simulink model "test"  (R2024b)
settings: Solver=VariableStepAuto  StartTime=0.0  StopTime=0.2  FixedStep=1e-6  RelTol=1e-3
libraries: spsMosfetLib x12, spsDiodeLib x6, spsSeriesRLCBranchLib x6, spsCurrentMeasurementLib x3, spsDCVoltageSourceLib x3, spsVoltageMeasurementLib x3, spsSeriesRLCLoadLib x1, spspowerguiLib x1
settings Model: Creator=medos  LastModifiedBy=medos
settings DataIOCC: InspectSignalLogs=on  ReturnWorkspaceOutputs=off

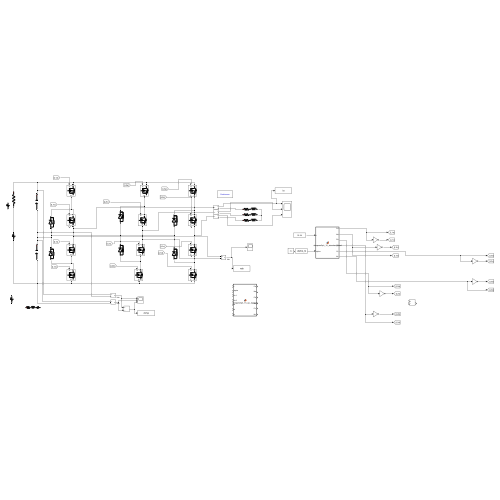
[thumbnail: Simulink's stored preview of the top-level diagram]
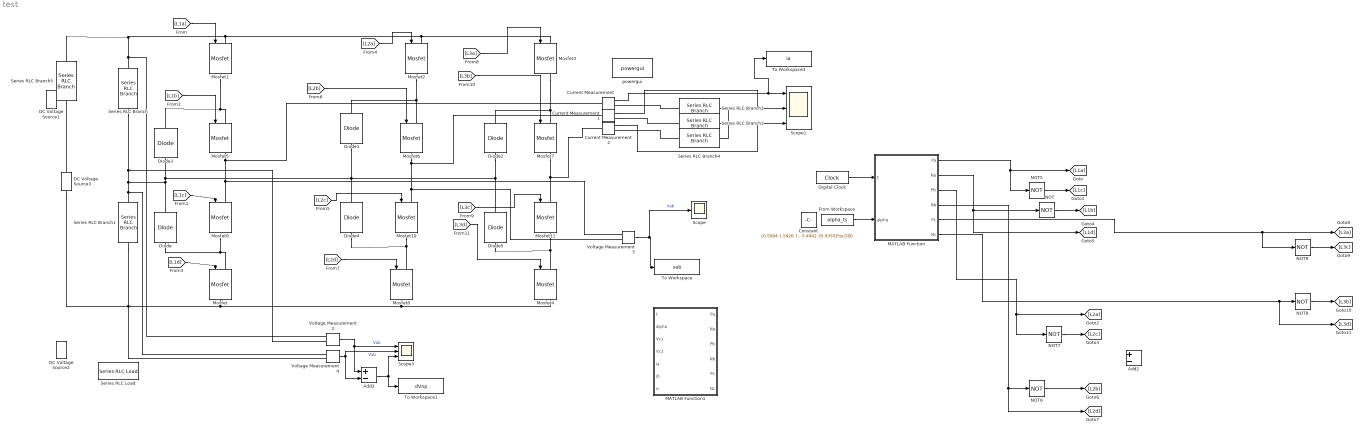
== system test ==
  Add2 : Sum  Inputs=+-
  Add3 : Sum  Inputs=+-
  Constant : Constant  Value="[0.5094\t1.5926\t7.8326\t9.5495\t13.4005\t15.2995\t15.5495\t16.5629\t19.0904\t22.9505\t24.7507\t29.3515\t30.4092\t35.4942\t35.9355]*pi/180"  SampleTime=-1
  Current Measurement : spsCurrentMeasurementLib/Current Measurement  PhasorSimulation=off  OutputType=Complex  PSBequivalent=0
  Current Measurement1 : spsCurrentMeasurementLib/Current Measurement  PhasorSimulation=off  OutputType=Complex  PSBequivalent=0
  Current Measurement2 : spsCurrentMeasurementLib/Current Measurement  PhasorSimulation=off  OutputType=Complex  PSBequivalent=0
  DC Voltage Source1 : spsDCVoltageSourceLib/DC Voltage Source  Amplitude=250  Measurements=None
  DC Voltage Source2 : spsDCVoltageSourceLib/DC Voltage Source  Amplitude=250  Measurements=None
  DC Voltage Source3 : spsDCVoltageSourceLib/DC Voltage Source  Amplitude=800  Measurements=None
  Digital Clock : DigitalClock  SampleTime=1e-6
  Diode{,1..5} (6 alike) : spsDiodeLib/Diode  Ron=0.001  Lon=0  Vf=0.8  IC=0  UseSnubber=0  Rs=500  Cs=250e-9  Measurements=off
  From Workspace : FromWorkspace  VariableName=alpha_ts  SampleTime=-1  Interpolate=off  OutputAfterFinalValue=Holding final value
  MATLAB Function : MATLAB Function  TreatAsAtomicUnit=on
  MATLAB Function1 : MATLAB Function  TreatAsAtomicUnit=on
  Mosfet{,1..2,6,8..10} (7 alike) : spsMosfetLib/Mosfet  Ron=0.1  Lon=0  Rd=0.01  Vfd=0  IC=0  Rs=1e5  Cs=inf  Measurements=off
  Mosfet{3..5,7,11} (5 alike) : spsMosfetLib/Mosfet  Ron=0.1  Lon=0  Rd=0.01  Vfd=0  IC=0  Rs=1e5  Cs=inf  Measurements=on
  NOT{,5..9} (6 alike) : Logic  Operator=NOT  IconShape=distinctive  AllPortsSameDT=off  OutDataTypeStr=boolean
  Scope : Scope
  Scope1 : Scope  NumInputPorts=3
  Scope3 : Scope  NumInputPorts=3
  Series RLC Branch : spsSeriesRLCBranchLib/Series RLC Branch  LConnTagsString=__new0  RConnTagsString=__new0  BranchType=C  Resistance=0.01  Inductance=1e-3  SetiL0=off  InitialCurrent=0  Capacitance=470e-6  Setx0=off  InitialVoltage=0  Measurements=None
  Series RLC Branch1 : spsSeriesRLCBranchLib/Series RLC Branch  LConnTagsString=__new0  RConnTagsString=__new0  BranchType=C  Resistance=0.01  Inductance=1e-3  SetiL0=off  InitialCurrent=0  Capacitance=470e-6  Setx0=off  InitialVoltage=0  Measurements=None
  Series RLC Branch2 : spsSeriesRLCBranchLib/Series RLC Branch  LConnTagsString=__new0  RConnTagsString=__new0  BranchType=RL  Resistance=64  Inductance=0.18  SetiL0=off  InitialCurrent=0  Capacitance=1e-6  Setx0=off  InitialVoltage=0  Measurements=None
  Series RLC Branch3 : spsSeriesRLCBranchLib/Series RLC Branch  LConnTagsString=__new0  RConnTagsString=__new0  BranchType=RL  Resistance=64  Inductance=0.18  SetiL0=off  InitialCurrent=0  Capacitance=1e-6  Setx0=off  InitialVoltage=0  Measurements=None
  Series RLC Branch4 : spsSeriesRLCBranchLib/Series RLC Branch  LConnTagsString=__new0  RConnTagsString=__new0  BranchType=RL  Resistance=64  Inductance=0.18  SetiL0=off  InitialCurrent=0  Capacitance=1e-6  Setx0=off  InitialVoltage=0  Measurements=None
  Series RLC Branch5 : spsSeriesRLCBranchLib/Series RLC Branch  LConnTagsString=__new0  RConnTagsString=__new0  BranchType=R  Resistance=0.0001  Inductance=1e-3  SetiL0=off  InitialCurrent=0  Capacitance=470e-6  Setx0=off  InitialVoltage=0  Measurements=None
  Series RLC Load : spsSeriesRLCLoadLib/Series RLC Load  LConnTagsString=a  RConnTagsString=__new0  NominalVoltage=1000  NominalFrequency=60  ActivePower=10e3  InductivePower=100  CapacitivePower=100  Setx0=off  InitialVoltage=0  SetiL0=off  InitialCurrent=0  Measurements=None  LoadType=constant Z
  To Workspace : ToWorkspace  VariableName=vab  SaveFormat=Timeseries  SampleTime=-1
  To Workspace1 : ToWorkspace  VariableName=dVnp  SaveFormat=Timeseries  SampleTime=-1
  To Workspace3 : ToWorkspace  VariableName=ia  SaveFormat=Timeseries  SampleTime=-1
  Voltage Measurement2 : spsVoltageMeasurementLib/Voltage Measurement  PhasorSimulation=off  OutputType=Complex  PSBequivalent=0
  Voltage Measurement3 : spsVoltageMeasurementLib/Voltage Measurement  PhasorSimulation=off  OutputType=Complex  PSBequivalent=0
  Voltage Measurement4 : spsVoltageMeasurementLib/Voltage Measurement  PhasorSimulation=off  OutputType=Complex  PSBequivalent=0
  powergui : spspowerguiLib/powergui  Priority=1  SimulationMode=Continuous  SampleTime=1e-6  frequency=50  Iterations=50  frequencyindice=0  Pbase=100e6  ErrMax=1e-4  UnitsV=kV  UnitsW=MW  buscounter=0  FunctionMessages=off  echomessages=off  EnableUseOfTLC=off  CurrentSourceSwitches=off  DisableSnubberDevices=off  DisableRonSwitches=off  DisableVfSwitches=off  DisplayEquations=off  AutomaticDiscreteSolvers=off  SolverType=Tustin/Backward Euler (TBE)  Interpol=off  ExternalGateDelay=off  methode=off  Ts=100  x0status=blocks  SPID=on  SwTol=0  HookPort=off  NonlinearTolerance=1e-4  nMaxIteration=100  ContinueOnMaxIteration=off  RestoreLinks=warning  ResistiveCurrentMeasurement=off  Frange=[0:2:500]  Ylog=off  Xlog=on  ShowGrid=off  save=off  variable=ZData  structure=0  ZoomFFT=off  StartTime=0.0  cycles=1  DisplayStyle=1  fundamental=60  FreqAxis=off  MaxFrequency=1000  frequencyindicesteady=1  RmsSteady=1  display=off
  wires:
  NOT8/1 -> [L3b]
  NOT5/1 -> [L1c]
  NOT9/1 -> [L3c]
  NOT/1 -> [L1b]
  NOT7/1 -> [L2c]
  NOT6/1 -> [L2b]
  [L1a] -> Mosfet1/1
  [L1c] -> Mosfet9/1
  [L1b] -> Mosfet5/1
  [L1d] -> Mosfet/1
  [L2a] -> Mosfet2/1
  [L2b] -> Mosfet6/1
  [L2c] -> Mosfet10/1
  [L2d] -> Mosfet8/1
  [L3a] -> Mosfet3/1
  [L3b] -> Mosfet7/1
  [L3c] -> Mosfet11/1
  [L3d] -> Mosfet4/1
  Voltage Measurement3/1 -> Scope/1, To Workspace/1  "Vab"
  Current Measurement/1 -> To Workspace3/1, Scope1/1
  Current Measurement1/1 -> Scope1/2
  Current Measurement2/1 -> Scope1/3
  Voltage Measurement2/1 -> Add3/1, Scope3/1  "Vab"
  Voltage Measurement4/1 -> Add3/2, Scope3/2  "Vab"
  Add3/1 -> Scope3/3, To Workspace1/1
  MATLAB Function/1(Pa) -> NOT5/1, [L1a]
  MATLAB Function/2(Na) -> NOT/1, [L1d]
  MATLAB Function/3(Pb) -> NOT7/1, [L2a]
  MATLAB Function/4(Nb) -> [L2d], NOT6/1
  MATLAB Function/5(Pc) -> NOT9/1, [L3a]
  MATLAB Function/6(Nc) -> NOT8/1, [L3d]
  Digital Clock/1 -> MATLAB Function/1(t)
  From Workspace/1 -> MATLAB Function/2(alpha)
  connections:
  Mosfet3/RConn1 -- Diode2/RConn1 -- Mosfet7/LConn1
  Mosfet7/RConn1 -- Mosfet11/LConn1 -- Current Measurement2/LConn1
  Mosfet11/RConn1 -- Diode5/LConn1 -- Mosfet4/LConn1
  Mosfet2/RConn1 -- Diode1/RConn1 -- Mosfet6/LConn1
  Mosfet6/RConn1 -- Voltage Measurement3/LConn2 -- Mosfet10/LConn1 -- Current Measurement1/LConn1
  Mosfet10/RConn1 -- Diode4/LConn1 -- Mosfet8/LConn1
  Mosfet1/RConn1 -- Diode3/RConn1 -- Mosfet5/LConn1
  Mosfet5/RConn1 -- Mosfet9/LConn1 -- Voltage Measurement3/LConn1 -- Current Measurement/LConn1
  Mosfet9/RConn1 -- Mosfet/LConn1 -- Diode/LConn1
  Mosfet/RConn1 -- Series RLC Branch1/RConn1 -- Voltage Measurement4/LConn2 -- DC Voltage Source3/LConn1 -- Mosfet8/RConn1 -- Mosfet4/RConn1
  Mosfet1/LConn1 -- Series RLC Branch5/LConn1 -- Voltage Measurement2/LConn1 -- Series RLC Branch/LConn1 -- Mosfet2/LConn1 -- Mosfet3/LConn1
  Series RLC Branch2/RConn1 -- Series RLC Branch4/RConn1 -- Series RLC Branch3/RConn1
  Diode/RConn1 -- Diode5/RConn1 -- Diode2/LConn1 -- Diode4/RConn1 -- Diode1/LConn1 -- Diode3/LConn1 -- Voltage Measurement4/LConn1 -- Series RLC Branch1/LConn1 -- Series RLC Branch/RConn1 -- Voltage Measurement2/LConn2
  Series RLC Branch2/LConn1 -- Current Measurement/RConn1
  Series RLC Branch3/LConn1 -- Current Measurement1/RConn1
  Series RLC Branch4/LConn1 -- Current Measurement2/RConn1
  DC Voltage Source3/RConn1 -- Series RLC Branch5/RConn1

== matlab function test/MATLAB Function1 ==
  data: t input; Pa output; alpha input; Na output; Pb output; Nb output; Pc output; Nc output; Vc1 input; Vc2 input; ia input; ib input; ic input
function [Pa, Na, Pb, Nb, Pc, Nc] = shmpwm3ph_15_np_balance(t, alpha, Vc1, Vc2, ia, ib, ic)
% SHMPWM with NP balancing using redundant zero-state selection
%
% Inputs:
%   t     : clock / simulation time
%   alpha : 15 switching angles (radians)
%   Vc1   : upper DC-link capacitor voltage
%   Vc2   : lower DC-link capacitor voltage
%   ia    : phase-a current
%   ib    : phase-b current
%   ic    : phase-c current
%
% Outputs:
%   Pa,Na,Pb,Nb,Pc,Nc : same P/N signals as your original function
%
% Gate mapping remains:
%   S1 = P
%   S2 = ~N
%   S3 = ~P
%   S4 = N
%
% Therefore for zero level:
%   P=0, N=0  -> [0 1 1 0]
%   P=1, N=1  -> [1 0 0 1]
%
% Assumption:
%   dVnp = Vc1 - Vc2
%   positive phase current means current flows from inverter to load
%
% If NP balancing acts in the wrong direction in your model,
% change npPolarity from +1 to -1.

alpha = sort(alpha(:)).';

f = 50;
w = 2*pi*f;

La = phase_level(w*t,          alpha);
Lb = phase_level(w*t - 2*pi/3, alpha);
Lc = phase_level(w*t - 4*pi/3, alpha);

% NP voltage error
dVnp = Vc1 - Vc2;

% Tuning parameters
Vband      = 1.0;    % dead-band in volts (try 1 to 3 V)
Imin       = 1e-3;   % current threshold to avoid noise around zero
npPolarity = -1;     % if behavior becomes worse, change to -1

[Pa, Na] = level_to_PN_np(La, dVnp, ia, Vband, Imin, npPolarity);
[Pb, Nb] = level_to_PN_np(Lb, dVnp, ib, Vband, Imin, npPolarity);
[Pc, Nc] = level_to_PN_np(Lc, dVnp, ic, Vband, Imin, npPolarity);

end


function L = phase_level(theta, alpha)

theta = mod(theta, 2*pi);

if theta <= pi/2
    L = first_quarter_level(theta, alpha);

elseif theta <= pi
    L = first_quarter_level(pi - theta, alpha);

elseif theta <= 3*pi/2
    L = -first_quarter_level(theta - pi, alpha);

else
    L = -first_quarter_level(2*pi - theta, alpha);
end

end


function L = first_quarter_level(theta, alpha)

L = 0;

for k = 1:length(alpha)
    if theta >= alpha(k)
        L = 1 - L;   % 0->1->0->1...
    else
        break;
    end
end

end


function [P, N] = level_to_PN_np(L, dVnp, iph, Vband, Imin, npPolarity)

% Positive level
if L > 0.5
    P = 1;
    N = 0;
    return;
end

% Negative level
if L < -0.5
    P = 0;
    N = 1;
    return;
end

% Zero level: choose between the two redundant zero states
%   P=0,N=0  -> [0 1 1 0]
%   P=1,N=1  -> [1 0 0 1]

% If imbalance is very small or current is too small, use default zero state
if abs(dVnp) < Vband || abs(iph) < Imin
    P = 0;
    N = 0;
    return;
end

% NP-balancing rule
% Assumption:
%   choose zero state based on sign(dVnp * iph)
%
% If this worsens the imbalance in your model,
% just flip npPolarity from +1 to -1.
if npPolarity * dVnp * iph >= 0
    P = 0;
    N = 0;
else
    P = 1;
    N = 1;
end

end

== matlab function test/MATLAB Function ==
  data: t input; Pa output; alpha input double size=[1 15]; Na output; Pb output; Nb output; Pc output; Nc output
function [Pa, Na, Pb, Nb, Pc, Nc] = shmpwm3ph_15_standard_fixed(t, alpha)

alpha = sort(alpha(:)).';

f = 50;
w = 2*pi*f;

La = phase_level(w*t,          alpha);
Lb = phase_level(w*t - 2*pi/3, alpha);
Lc = phase_level(w*t - 4*pi/3, alpha);

[Pa, Na] = level_to_PN(La);
[Pb, Nb] = level_to_PN(Lb);
[Pc, Nc] = level_to_PN(Lc);

end


function L = phase_level(theta, alpha)

theta = mod(theta, 2*pi);

if theta <= pi/2
    L = first_quarter_level(theta, alpha);

elseif theta <= pi
    L = first_quarter_level(pi - theta, alpha);

elseif theta <= 3*pi/2
    L = -first_quarter_level(theta - pi, alpha);

else
    L = -first_quarter_level(2*pi - theta, alpha);
end

end


function L = first_quarter_level(theta, alpha)

% IMPORTANT:
% Standard waveform from the paper starts at 0 in the first quarter,
% then toggles 0/1 at every switching angle.
L = 0;

for k = 1:length(alpha)
    if theta >= alpha(k)
        L = 1 - L;   % toggle: 0->1->0->1...
    else
        break;
    end
end

end


function [P, N] = level_to_PN(L)

if L > 0.5
    P = 1; N = 0;
elseif L < -0.5
    P = 0; N = 1;
else
    P = 0; N = 0;
end

end
